simulink model "impmodel"  (R2023a)
settings: Solver=FixedStepDiscrete  StartTime=0.0  StopTime=8  RelTol=1e-3  EnableMultiTasking=on
values from neighbouring files (symbols this model uses):
  availableSpeedModes = 3    [params_f2838.mat]
  inverter_DRV8300 =     [params_f2838.mat]
  PI_params =     [params_f2838.mat]
  pmsm_ECI6360 =     [params_f2838.mat]
  PU_System =     [params_f2838.mat]
  target_f2838 =     [params_f2838.mat]
  Ts = 5e-05    [params_f2838.mat]
  Ts_motor = 2.5e-05    [params_f2838.mat]
  Ts_simulink = 2.5e-05    [params_f2838.mat]
  Ts_speed = 0.0005    [params_f2838.mat]
undefined symbols (not defined in the file or in its folder): Down, GPTRIP1SEL, TZ1, Up
libraries: simulink x35, c2802xlib x11, idelinklib_common x8, procinterlib x8, mcbcontrolslib x8, c280xlib x7, mcbpositiondecoderlib x7, slpidlib x5, svdschedulerlib x4, c2838xlib x2, autolibpmsminterior x1, mcbplantlib x1
(part 2 of 4)

== system impmodel/Input Controller/SpeedCommand_CodeGen ==
  note: This Subsystem is essential due to the fact that the voltage at the potentiometer will not reach 3.3 V.
      | At an ADC value bigger than 4000 the output will jump to 4095 (full speed)
  ADC1 : c2802xlib/ADC  blkParamProc=C2000_Type4  ADCModule=A  samplingMode=Single sample mode  ADCResolution=12-bit (Single-ended input)  useSOC1=SOC2  useSOC2=SOC0_SOC1  SOCAcquisitionWindow=7  SOCTriggerSource=Software  SOCInterruptTrigger=No ADCINT  Ts=0.01  dType=uint16  postInterrupt=off  interruptSel=ADCINT1  ADCINTContinuous=on  endma=off  chdma=1  conv1=ADCINA0  conv2=ADCINA0 and ADCINB0  conv1_Type4=ADCIN0  conv2_Type4=ADCIN0 and ADCIN1
      settings: LibrarySourceBlock=c2838xlib/ADC
  Check for SpeedRef : Subsystem
  normalizeADCValue : Gain  Gain=1/4095  OutDataTypeStr=fixdt(1,32,17)  RndMeth=Ceiling
  Speed_Ref : Outport
  wires:
  normalizeADCValue/1 -> Speed_Ref/1
  Check for SpeedRef/1(Out1) -> normalizeADCValue/1
  ADC1/1 -> Check for SpeedRef/1(In1)

== system impmodel/Input Controller/Subsystem ==
  ADC1 : c2802xlib/ADC  blkParamProc=C2000_Type4  ADCModule=C  samplingMode=Single sample mode  ADCResolution=12-bit (Single-ended input)  useSOC1=SOC5  useSOC2=SOC0_SOC1  SOCAcquisitionWindow=15  SOCTriggerSource=Software  SOCInterruptTrigger=No ADCINT  Ts=0.2  dType=uint16  postInterrupt=off  interruptSel=ADCINT1  ADCINTContinuous=on  endma=off  chdma=1  conv1=ADCINA0  conv2=ADCINA0 and ADCINB0  conv1_Type4=ADCIN2  conv2_Type4=ADCIN0 and ADCIN1
      settings: LibrarySourceBlock=c2838xlib/ADC
  Constant2 : Constant  Value=500e-3  OutDataTypeStr=fixdt(1,32,17)  SampleTime=-1
  Constant3 : Constant  Value=0.01  OutDataTypeStr=fixdt(1,32,17)  SampleTime=-1
  Divide : Product  Inputs=*/  OutDataTypeStr=fixdt(1,32,17)
  Gain : Gain  Gain=3.3/4095  OutDataTypeStr=fixdt(1,32,17)
  Subtract1 : Sum  Inputs=+-  OutDataTypeStr=fixdt(1,32,17)
  TCP_temp : Subsystem
  temperatureMOS : Outport
  wires:
  Constant3/1 -> Divide/2
  Gain/1 -> Subtract1/1
  Divide/1 -> TCP_temp/1(In1), temperatureMOS/1
  Constant2/1 -> Subtract1/2
  Subtract1/1 -> Divide/1
  ADC1/1 -> Gain/1

== system impmodel/Input Controller/speedMode_CodeGen ==
  Data Type Conversion : DataTypeConversion  OutDataTypeStr=fixdt(1,32,17)  SaturateOnIntegerOverflow=off  RndMeth=Floor
  Select first element : Selector  InputPortWidth=4  IndexOptions=Index vector (dialog)  Indices=[1]  OutputSizes=1
  Terminator : Terminator
  eCAN Receive1 : c280xlib/eCAN Receive  chipFamily=C280x  useModule=eCAN_A  mailboxNo=15  messageID=hex2dec('102')  messageType=Standard (11-bit identifier)  enableAcceptanceFiltering=off  messageIDMask=0  sampleTime=0.2  dataType=uint16  outputAction=Output last received values  initValue=0  outputMessageID=off  outputMessageLength=off  outputMessageTimeStamp=off  postInterrupt=off  interruptLine=0
      settings: LibrarySourceBlock=c28004xlib/eCAN Receive
  limit modes between 1 and 'availableSpeedModes' : Saturate  UpperLimit=availableSpeedModes  LowerLimit=1
  speedMode_CodeGen : Outport
  wires:
  eCAN Receive1/2 -> Select first element/1
  eCAN Receive1/1 -> Terminator/1
  Select first element/1 -> Data Type Conversion/1
  Data Type Conversion/1 -> limit modes between 1 and 'availableSpeedModes'/1
  limit modes between 1 and 'availableSpeedModes'/1 -> speedMode_CodeGen/1

== system impmodel/Inverter and Motor - Plant Model/Codegeneration ==
  Duty_Cycles : Inport
  Ground : Ground
  Ground1 : Ground
  Terminator : Terminator
  Iab_fb_Sim : Outport  VectorParamsAs1DForOutWhenUnconnected=off
  Pos_fb_Sim : Outport  Port=2  VectorParamsAs1DForOutWhenUnconnected=off
  wires:
  Duty_Cycles/1 -> Terminator/1
  Ground/1 -> Iab_fb_Sim/1
  Ground1/1 -> Pos_fb_Sim/1

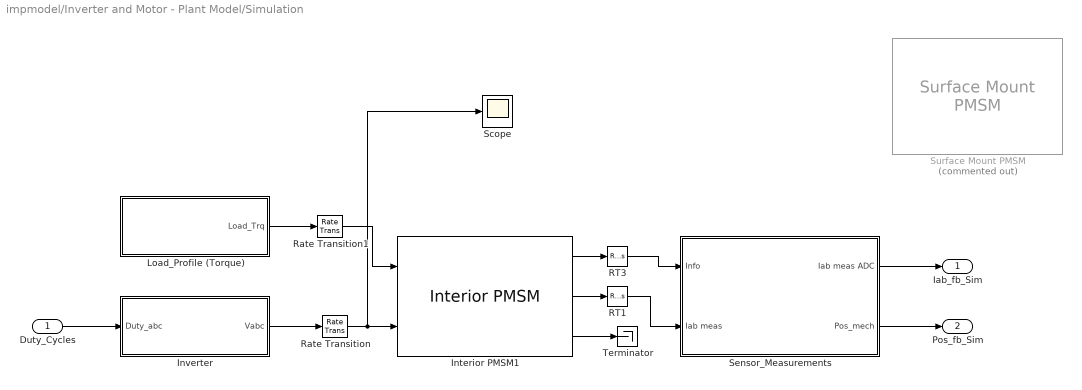
== system impmodel/Inverter and Motor - Plant Model/Simulation ==
  Duty_Cycles : Inport
  Interior PMSM1 : autolibpmsminterior/Interior PMSM  port_config=Torque  sim_type=Discrete  Ts=Ts_motor  P=pmsm_ECI6360.p  Rs=pmsm_ECI6360.Rs  Ldq=[pmsm_ECI6360.Ld, pmsm_ECI6360.Lq]  KConstText=Permanent flux linkage constant (lambda_pm):  lambda_pm=pmsm_ECI6360.FluxPM  Ke=pmsm_ECI6360.Ke  mechanical=[pmsm_ECI6360.J,0,0]  idq0=[0 0]  theta_init=0  omega_init=0  KConst=pmsm_ECI6360.FluxPM  lambda_pm_calc=pmsm_ECI6360.FluxPM  Kt=0.07  RefBlkName='autolibpmsminterior/Interior PMSM'  aMode=5
      settings: LibrarySourceBlock=mcblib/Electrical Systems/Motors/Interior PMSM
  Inverter : Subsystem
  Load_Profile (Torque) : Subsystem
  RT1 : RateTransition  Deterministic=off  OutPortSampleTime=Ts_simulink
  RT3 : RateTransition  Deterministic=off  OutPortSampleTime=Ts_simulink
  Rate Transition : RateTransition  Deterministic=off  OutPortSampleTime=Ts_motor
  Rate Transition1 : RateTransition  Deterministic=off  OutPortSampleTime=Ts_motor
  Scope : Scope
  Sensor_Measurements : Subsystem
  Surface Mount PMSM : autolibpmsmexterior/Surface Mount PMSM  Commented=on  port_config=Torque  sim_type=Discrete  Ts=Ts_motor  P=4  Rs=1  Ldq_=pmsm_ECI6360.Ld  KConstText=Permanent flux linkage constant (lambda_pm):  lambda_pm=0.039  Ke=pmsm_ECI6360.Ke  Kt=1.323  mechanical=[pmsm_ECI6360.J, pmsm_ECI6360.B, 0]  idq0=[0 0]  theta_init=0  omega_init=0  KConst=0.039  lambda_pm_calc=0.039  RefBlkName='autolibpmsmexterior/Surface Mount PMSM'  aMode=5  Ldq="[0.0002      0.0002]"
  Terminator : Terminator
  Iab_fb_Sim : Outport  VectorParamsAs1DForOutWhenUnconnected=off
  Pos_fb_Sim : Outport  Port=2  VectorParamsAs1DForOutWhenUnconnected=off
  wires:
  Sensor_Measurements/1(Iab meas ADC) -> Iab_fb_Sim/1
  Sensor_Measurements/2(Pos_mech) -> Pos_fb_Sim/1
  RT3/1 -> Sensor_Measurements/1(Info)
  Rate Transition1/1 -> Interior PMSM1/1
  RT1/1 -> Sensor_Measurements/2(Iab meas)
  Load_Profile (Torque)/1(Load_Trq) -> Rate Transition1/1
  Interior PMSM1/1 -> RT3/1
  Interior PMSM1/2 -> RT1/1
  Interior PMSM1/3 -> Terminator/1
  Rate Transition/1 -> Scope/1, Interior PMSM1/2
  Duty_Cycles/1 -> Inverter/1(Duty_abc)
  Inverter/1(Vabc) -> Rate Transition/1

== system impmodel/Speed Control/Digital_Freemode_Check ==
  Undervoltage_Sig : Inport
  Freemode : Inport  Port=2
  hot_temp : Inport  Port=3
  Check if Freemode is enabled : simulink/Logic and Bit Operations/Compare To Constant  relop===  const=1  OutDataTypeStr=boolean
  Check if MOSFETs are too hot : simulink/Logic and Bit Operations/Compare To Constant  relop===  const=1  OutDataTypeStr=boolean
  Check if Undervoltage is achieved : simulink/Logic and Bit Operations/Compare To Constant  relop===  const=1  OutDataTypeStr=boolean
  OR : Logic  Operator=OR  Inputs=3  AllPortsSameDT=off  OutDataTypeStr=boolean
  "Freemode_Sig  " : Outport
  wires:
  Freemode/1 -> Check if Freemode is enabled/1
  Undervoltage_Sig/1 -> Check if Undervoltage is achieved/1
  Check if Undervoltage is achieved/1 -> OR/1
  Check if Freemode is enabled/1 -> OR/2
  hot_temp/1 -> Check if MOSFETs are too hot/1
  Check if MOSFETs are too hot/1 -> OR/3
  OR/1 -> "Freemode_Sig  "/1

== system impmodel/Speed Control/Mechanical_Freemode_Check ==
  Freemode_Sig_Dig : Inport
  SafeState : Inport  Port=2
  If : If  IfExpression=u1 ~= 1
  If Action Subsystem : Subsystem  TreatAsAtomicUnit=on
  If Action Subsystem1 : Subsystem  TreatAsAtomicUnit=on
  Merge : Merge
  Freemode_Sig : Outport
  wires:
  SafeState/1 -> If/1
  Merge/1 -> Freemode_Sig/1
  Freemode_Sig_Dig/1 -> If Action Subsystem1/1(Freemode_Sig_Dig)
  If Action Subsystem/1(Out1) -> Merge/1
  If/1 -> If Action Subsystem/Action
  If Action Subsystem1/1(Out1) -> Merge/2
  If/2 -> If Action Subsystem1/Action

== system impmodel/Speed Control/PI_Controller_Speed ==
  N_ref : Inport
  N_fb : Inport  Port=2
  "  FreemodeEnabled?" : Inport  Port=3
  "Essential, so error of PI controller isn't rising" : Switch  Criteria=u2 > Threshold  OutDataTypeStr=fixdt(1,32,17)  SaturateOnIntegerOverflow=off  InputSameDT=off
  PID Controller : slpidlib/PID Controller  Controller=PI  Form=Parallel  TimeDomain=Discrete-time  UseExternalTs=off  SampleTime=-1  IntegratorMethod=Forward Euler  FilterMethod=Forward Euler  ControllerParametersSource=internal  P=PI_params.Kp_speed  I=PI_params.Ki_speed_texas*Ts_speed  UseKiTs=on  D=0  N=100  UseFilter=on  TunerSelectOption=Transfer Function Based (PID Tuner App)  InitialConditionSource=internal  InitialConditionForIntegrator=0  InitialConditionForFilter=0  DifferentiatorICPrevScaledInput=0  ExternalReset=none  TrackingMode=off  Kt=1  LimitOutput=on  SatLimitsSource=internal  UpperSaturationLimit=1  LowerSaturationLimit=-0.5  LinearizeAsGain=on  AntiWindupMode=clamping  Kb=1  LimitIntegrator=off  UpperIntegratorSaturationLimit=inf  LowerIntegratorSaturationLimit=-inf  RndMeth=Nearest  POutMin=[]  POutMax=[]  IOutMin=[]  IOutMax=[]  DOutMin=[]  DOutMax=[]  NOutMin=[]  NOutMax=[]  SumOutMin=[]  SumOutMax=[]  SaturationOutMin=[]  SaturationOutMax=[]  PParamMin=[]  PParamMax=[]  IParamMin=[]  IParamMax=[]  DParamMin=[]  DParamMax=[]  NParamMin=[]  NParamMax=[]  KbParamMin=[]  KbParamMax=[]  KtParamMin=[]  KtParamMax=[]  KbOutMin=[]  KbOutMax=[]  KtOutMin=[]  KtOutMax=[]  IntegratorOutMin=[]  IntegratorOutMax=[]  FilterOutMin=[]  FilterOutMax=[]  SumI1OutMin=[]  SumI1OutMax=[]  SumI2OutMin=[]  SumI2OutMax=[]  SumI3OutMin=[]  SumI3OutMax=[]  SumI4OutMin=[]  SumI4OutMax=[]  SumDOutMin=[]  SumDOutMax=[]  DifferentiatorOutMin=[]  DifferentiatorOutMax=[]  FilterDiffOutCoefMin=[]  FilterDiffOutCoefMax=[]  ReciprocalOutMin=[]  ReciprocalOutMax=[]  SumDenOutMin=[]  SumDenOutMax=[]  SumNumOutMin=[]  SumNumOutMax=[]  DivideOutMin=[]  DivideOutMax=[]  UdiffTsProdOutMin=[]  UdiffTsProdOutMax=[]  NTsProdOutMin=[]  NTsProdOutMax=[]  UintegralTsProdOutMin=[]  UintegralTsProdOutMax=[]  UngainTsProdOutMin=[]  UngainTsProdOutMax=[]  ClampingZeroOutDataTypeStr=Inherit: Inherit via back propagation  ClampingZeroOutMin=[]  ClampingZeroOutMax=[]  FilterDenConstantOutDataTypeStr=Inherit: Inherit via back propagation  FilterDenConstantOutMin=[]  FilterDenConstantOutMax=[]  PCopyOutDataTypeStr=Inherit: Inherit via back propagation  PCopyOutMin=[]  PCopyOutMax=[]  NCopyOutDataTypeStr=Inherit: Inherit via back propagation  NCopyOutMin=[]  NCopyOutMax=[]  IntegratorContinuousStateAttributes=''  IntegratorStateMustResolveToSignalObject=off  IntegratorRTWStateStorageClass=Auto  FilterContinuousStateAttributes=''  FilterStateMustResolveToSignalObject=off  FilterRTWStateStorageClass=Auto  ParallelPVariant=InternalParameters  IdealPVariant=Disabled  IVariant=InternalParameters  DVariant=Disabled  IntegratorVariant=Discrete  SatVariant=Enabled  AWVariant=DiscClampingParallel  PCopyVariant=Disabled  TRVariant=Disabled  FdbkBlocksVariant=Forward  IdealPFdbkVariant=Disabled  SatFdbkVariant=Disabled  DerivativeFilterVariant=Disabled  NVariant=Disabled  NCopyVariant=Disabled_SignalSpec  FilterICVariant=Disabled  IntegratorICVariant=InternalICs  ExternalResetVariant=Disabled  TRSumVariant=Passthrough  SumFdbkVariant=Disabled  SumVariant=Sum_PI  TsampFilterVariant=InternalTs  TsampNgainVariant=Passthrough  TsampIntegralVariant=Disabled_SignalSpec  ExternalSaturationOutDataTypeStr=Inherit: Same as second input
  Saturation : Saturate  UpperLimit=0  LowerLimit=0
  Sum : Sum  Inputs=|+-  RndMeth=Round
  Iq_ref : Outport  VectorParamsAs1DForOutWhenUnconnected=off
  wires:
  N_ref/1 -> Saturation/1, "Essential, so error of PI controller isn't rising"/3
  N_fb/1 -> Sum/2
  PID Controller/1 -> Iq_ref/1
  "  FreemodeEnabled?"/1 -> "Essential, so error of PI controller isn't rising"/2
  Saturation/1 -> "Essential, so error of PI controller isn't rising"/1
  Sum/1 -> PID Controller/1
  "Essential, so error of PI controller isn't rising"/1 -> Sum/1

== system impmodel/Speed Control/Speed calculator ==
  Speed_Ref_PU : Inport
  speedMode : Inport  Port=2
  Gain : Gain  Gain=floor(PU_System.N_base/availableSpeedModes)  OutDataTypeStr=fixdt(1,32,17)  RndMeth=Ceiling
  Product : Product  OutDataTypeStr=fixdt(1,32,17)
  Subsystem : Subsystem  Commented=through
  rpm2PU : Gain  Gain=1/PU_System.N_base  OutMax=1  OutDataTypeStr=fixdt(1,32,17)
  N_Ref : Outport
  wires:
  Speed_Ref_PU/1 -> Gain/1
  Gain/1 -> Product/2
  speedMode/1 -> Product/1
  Product/1 -> rpm2PU/1
  rpm2PU/1 -> Subsystem/1(In1)
  Subsystem/1(Out1) -> N_Ref/1

== system impmodel/Speed Control/TCP_SpeedRef ==
  In1 : Inport
  Data_Type_Fixed_Point : Subsystem  VariantControl=~isequal(dataType,'single')
  Interprocess Data Write : procinterlib/Interprocess Data Write  showPort=off  ChannelNum=6  NumBuff=1  IsIntEnabled=1  EnInterrupt=on  IPCBetween=1  CurrentPU=0  DataType=uint8  PartCores=CPU1<->CM  TargetType=0  ClientPU=TriCore1  ClientIntPrio=50
  wires:
  Data_Type_Fixed_Point/1(Data_Log) -> Interprocess Data Write/1
  In1/1 -> Data_Type_Fixed_Point/1(In1)

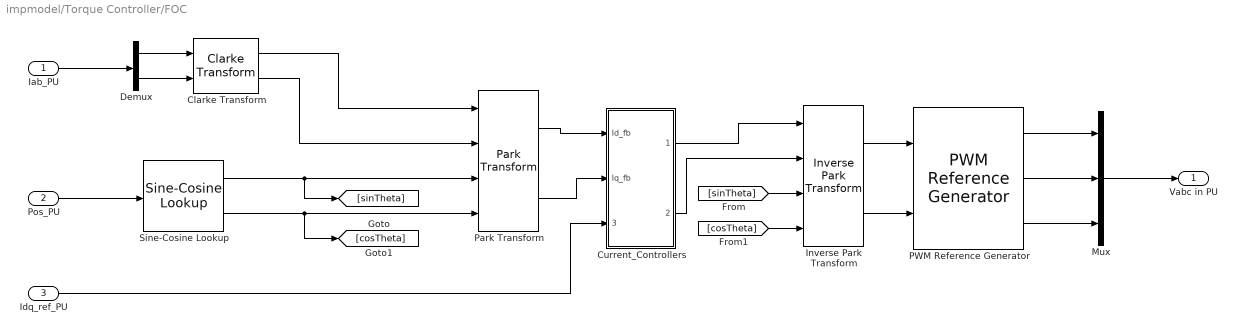
== system impmodel/Torque Controller/FOC ==
  Iab_PU : Inport
  Pos_PU : Inport  Port=2
  Idq_ref_PU : Inport  Port=3
  Clarke Transform : mcbcontrolslib/Clarke Transform  VariantControl=Variant2
      settings: LibrarySourceBlock=mcbhdllib/Controls/Math Transforms/Clarke Transform
  Current_Controllers : Subsystem
  Demux : Demux  Outputs=2
  Inverse Park Transform : mcbcontrolslib/Inverse Park Transform  AxisAlignment=D-axis
      settings: LibrarySourceBlock=mcbhdllib/Controls/Math Transforms/Inverse Park Transform
  Mux : Mux  Inputs=3
  PWM Reference Generator : mcbcontrolslib/PWM Reference Generator  inSignal=Valphabeta  modType=SVM: space vector modulation
      settings: LibrarySourceBlock=mcblib/Controls/Math Transforms/PWM Reference Generator
  Park Transform : mcbcontrolslib/Park Transform  AxisAlignment=D-axis
      settings: LibrarySourceBlock=mcbhdllib/Controls/Math Transforms/Park Transform
  Sine-Cosine Lookup : mcbcontrolslib/Sine-Cosine Lookup  AngleInput=Per-unit  N_points=1024
      settings: LibrarySourceBlock=mcblib/Controls/Math Transforms/Sine-Cosine Lookup
  Vabc in PU : Outport
  wires:
  Iab_PU/1 -> Demux/1
  Demux/1 -> Clarke Transform/1
  Demux/2 -> Clarke Transform/2
  Clarke Transform/1 -> Park Transform/1
  Clarke Transform/2 -> Park Transform/2
  Sine-Cosine Lookup/1 -> [sinTheta], Park Transform/3
  Sine-Cosine Lookup/2 -> [cosTheta], Park Transform/4
  Park Transform/1 -> Current_Controllers/1(Id_fb)
  Park Transform/2 -> Current_Controllers/2(Iq_fb)
  Idq_ref_PU/1 -> Current_Controllers/3(Idq_ref_PU)
  [sinTheta] -> Inverse Park Transform/3
  [cosTheta] -> Inverse Park Transform/4
  Inverse Park Transform/1 -> PWM Reference Generator/1
  Inverse Park Transform/2 -> PWM Reference Generator/2
  PWM Reference Generator/1 -> Mux/1
  PWM Reference Generator/2 -> Mux/2
  PWM Reference Generator/3 -> Mux/3
  Mux/1 -> Vabc in PU/1
  Pos_PU/1 -> Sine-Cosine Lookup/1
  Current_Controllers/1(Vd_ref) -> Inverse Park Transform/1
  Current_Controllers/2(Vq_ref) -> Inverse Park Transform/2

== system impmodel/Torque Controller/Iab_Meas_ADC ==
  ADC : c2802xlib/ADC  blkParamProc=C2000_Type4  ADCModule=B  samplingMode=Single sample mode  ADCResolution=12-bit (Single-ended input)  useSOC1=SOC0  useSOC2=SOC0_SOC1  SOCAcquisitionWindow=13  SOCTriggerSource=ePWM6_ADCSOCA  SOCInterruptTrigger=No ADCINT  Ts=-1  dType=uint16  postInterrupt=off  interruptSel=ADCINT1  ADCINTContinuous=on  endma=off  chdma=1  conv1=ADCINA0  conv2=ADCINA0 and ADCINB0  conv1_Type4=ADCIN0  conv2_Type4=ADCIN0 and ADCIN1
      settings: LibrarySourceBlock=c2838xlib/ADC
  ADC1 : c2802xlib/ADC  blkParamProc=C2000_Type4  ADCModule=B  samplingMode=Single sample mode  ADCResolution=12-bit (Single-ended input)  useSOC1=SOC1  useSOC2=SOC0_SOC1  SOCAcquisitionWindow=13  SOCTriggerSource=ePWM6_ADCSOCA  SOCInterruptTrigger=No ADCINT  Ts=-1  dType=uint16  postInterrupt=on  interruptSel=ADCINT1  ADCINTContinuous=on  endma=off  chdma=1  conv1=ADCINA0  conv2=ADCINA0 and ADCINB0  conv1_Type4=ADCIN2  conv2_Type4=ADCIN0 and ADCIN1
      settings: LibrarySourceBlock=c2838xlib/ADC
  Mux : Mux  Inputs=2
  Iab_ADC : Outport
  wires:
  Mux/1 -> Iab_ADC/1
  ADC/1 -> Mux/1
  ADC1/1 -> Mux/2

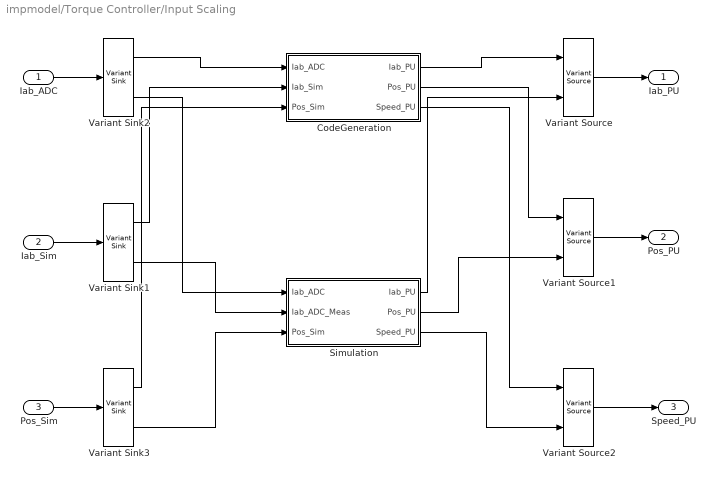
== system impmodel/Torque Controller/Input Scaling ==
  Iab_ADC : Inport
  Iab_Sim : Inport  Port=2
  Pos_Sim : Inport  Port=3
  CodeGeneration : Subsystem
  Simulation : Subsystem
  Variant Sink1 : VariantSink  VariantControlMode=sim codegen switching
  Variant Sink2 : VariantSink  VariantControlMode=sim codegen switching
  Variant Sink3 : VariantSink  VariantControlMode=sim codegen switching
  Variant Source : VariantSource  VariantControlMode=sim codegen switching
  Variant Source1 : VariantSource  VariantControlMode=sim codegen switching
  Variant Source2 : VariantSource  VariantControlMode=sim codegen switching
  Iab_PU : Outport
  Pos_PU : Outport  Port=2
  Speed_PU : Outport  Port=3
  wires:
  Pos_Sim/1 -> Variant Sink3/1
  Iab_Sim/1 -> Variant Sink1/1
  Iab_ADC/1 -> Variant Sink2/1
  Variant Sink2/1 -> CodeGeneration/1(Iab_ADC)
  Variant Sink1/1 -> CodeGeneration/2(Iab_Sim)
  Variant Sink3/1 -> CodeGeneration/3(Pos_Sim)
  Variant Sink2/2 -> Simulation/1(Iab_ADC)
  Variant Sink1/2 -> Simulation/2(Iab_ADC_Meas)
  Variant Sink3/2 -> Simulation/3(Pos_Sim)
  CodeGeneration/1(Iab_PU) -> Variant Source/1
  Simulation/1(Iab_PU) -> Variant Source/2
  CodeGeneration/2(Pos_PU) -> Variant Source1/1
  Simulation/2(Pos_PU) -> Variant Source1/2
  Simulation/3(Speed_PU) -> Variant Source2/2
  CodeGeneration/3(Speed_PU) -> Variant Source2/1
  Variant Source/1 -> Iab_PU/1
  Variant Source1/1 -> Pos_PU/1
  Variant Source2/1 -> Speed_PU/1

== system impmodel/Torque Controller/Output ==
  Scaled_DC : Inport
  CodeGeneration : Subsystem
  Scope : Scope
  Simulation : Subsystem
  Variant Sink : VariantSink  VariantControlMode=sim codegen switching
  Duty Cycle : Outport
  wires:
  Scaled_DC/1 -> Variant Sink/1
  Simulation/1(Output) -> Scope/1, Duty Cycle/1
  Variant Sink/1 -> CodeGeneration/1(In1)
  Variant Sink/2 -> Simulation/1(Input)

== system impmodel/Torque Controller/PWM1 ==
  Scaled_DC_PWM1 : Inport
  Freemode_Sig : Inport  Port=2
  Constant : Constant  Value=0  OutDataTypeStr=fixdt(1,32,17)  SampleTime=-1
  Constant1 : Constant  OutDataTypeStr=fixdt(1,32,17)  SampleTime=-1
  Switch : Switch  Criteria=u2 > Threshold  SaturateOnIntegerOverflow=off  InputSameDT=off  OutDataTypeStr=Inherit: Same as first input
  Switch1 : Switch  Criteria=u2 > Threshold  SaturateOnIntegerOverflow=off  InputSameDT=off  OutDataTypeStr=Inherit: Same as first input
  WA : Outport
  WB : Outport  Port=2
  wires:
  Freemode_Sig/1 -> Switch1/2, Switch/2
  Switch/1 -> WA/1
  Switch1/1 -> WB/1
  Scaled_DC_PWM1/1 -> Switch/3, Switch1/3
  Constant/1 -> Switch/1
  Constant1/1 -> Switch1/1

== system impmodel/Torque Controller/PWM2 ==
  Scaled_DC_PWM2 : Inport
  Freemode_Sig : Inport  Port=2
  Constant : Constant  Value=0  OutDataTypeStr=fixdt(1,32,17)  SampleTime=-1
  Constant1 : Constant  OutDataTypeStr=fixdt(1,32,17)  SampleTime=-1
  Switch : Switch  Criteria=u2 > Threshold  SaturateOnIntegerOverflow=off  InputSameDT=off  OutDataTypeStr=Inherit: Same as first input
  Switch1 : Switch  Criteria=u2 > Threshold  SaturateOnIntegerOverflow=off  InputSameDT=off  OutDataTypeStr=Inherit: Same as first input
  WA : Outport
  WB : Outport  Port=2
  wires:
  Switch/1 -> WA/1
  Switch1/1 -> WB/1
  Constant/1 -> Switch/1
  Freemode_Sig/1 -> Switch/2, Switch1/2
  Constant1/1 -> Switch1/1
  Scaled_DC_PWM2/1 -> Switch1/3, Switch/3

== system impmodel/Torque Controller/PWM3 ==
  Scaled_DC_PWM3 : Inport
  Freemode_Sig : Inport  Port=2
  Constant : Constant  Value=0  OutDataTypeStr=fixdt(1,32,17)  SampleTime=-1
  Constant1 : Constant  OutDataTypeStr=fixdt(1,32,17)  SampleTime=-1
  Switch : Switch  Criteria=u2 > Threshold  SaturateOnIntegerOverflow=off  InputSameDT=off  OutDataTypeStr=Inherit: Same as first input
  Switch1 : Switch  Criteria=u2 > Threshold  SaturateOnIntegerOverflow=off  InputSameDT=off  OutDataTypeStr=Inherit: Same as first input
  WA : Outport
  WB : Outport  Port=2
  wires:
  Switch/1 -> WA/1
  Switch1/1 -> WB/1
  Constant/1 -> Switch/1
  Freemode_Sig/1 -> Switch1/2, Switch/2
  Constant1/1 -> Switch1/1
  Scaled_DC_PWM3/1 -> Switch1/3, Switch/3

== system impmodel/Torque Controller/Scaling DutyCycles ==
  Unscaled_DC : Inport
  CodeGen : Subsystem
  Demux : Demux  Outputs=3
  Sim : Subsystem
  Variant Sink : VariantSink  VariantControlMode=sim codegen switching
  Variant Source : VariantSource  VariantControlMode=sim codegen switching
  Scaled_DC_PWM1 : Outport
  Scaled_DC_PWM2 : Outport  Port=2
  Scaled_DC_PWM3 : Outport  Port=3
  wires:
  Demux/1 -> Scaled_DC_PWM1/1
  Demux/2 -> Scaled_DC_PWM2/1
  Demux/3 -> Scaled_DC_PWM3/1
  Variant Source/1 -> Demux/1
  Unscaled_DC/1 -> Variant Sink/1
  Sim/1(Out1) -> Variant Source/2
  Variant Sink/2 -> Sim/1(In1)
  Variant Sink/1 -> CodeGen/1(In1)
  CodeGen/1(Out1) -> Variant Source/1

== system impmodel/Torque Controller/TCP_Position ==
  In1 : Inport
  Data_Type_Fixed_Point : Subsystem  VariantControl=~isequal(dataType,'single')
  Interprocess Data Write : procinterlib/Interprocess Data Write  showPort=off  ChannelNum=0  NumBuff=1  IsIntEnabled=1  EnInterrupt=on  IPCBetween=1  CurrentPU=0  DataType=uint8  PartCores=CPU1<->CM  TargetType=0  ClientPU=TriCore1  ClientIntPrio=50
  wires:
  Data_Type_Fixed_Point/1(Data_Log) -> Interprocess Data Write/1
  In1/1 -> Data_Type_Fixed_Point/1(In1)

== system impmodel/Torque Controller/TCP_Speed ==
  " " : Inport
  Data_Type_Fixed_Point : Subsystem  VariantControl=~isequal(dataType,'single')
  Interprocess Data Write : procinterlib/Interprocess Data Write  showPort=off  ChannelNum=1  NumBuff=1  IsIntEnabled=1  EnInterrupt=on  IPCBetween=1  CurrentPU=0  DataType=uint8  PartCores=CPU1<->CM  TargetType=0  ClientPU=TriCore1  ClientIntPrio=50
  wires:
  Data_Type_Fixed_Point/1(Data_Log) -> Interprocess Data Write/1
  " "/1 -> Data_Type_Fixed_Point/1(In1)

== system impmodel/ADC Offset Function/Calculate ADC Offset /For Iterator Subsystem ==
  ADC_B_IN0 : c2802xlib/ADC  Priority=20  blkParamProc=C2000_Type4  ADCModule=B  samplingMode=Single sample mode  ADCResolution=12-bit (Single-ended input)  useSOC1=SOC2  useSOC2=SOC0_SOC1  SOCAcquisitionWindow=15  SOCTriggerSource=Software  SOCInterruptTrigger=No ADCINT  Ts=-1  dType=uint16  postInterrupt=off  interruptSel=ADCINT1  ADCINTContinuous=on  endma=off  chdma=1  conv1=ADCINA0  conv2=ADCINA0 and ADCINB0  conv1_Type4=ADCIN0  conv2_Type4=ADCIN0 and ADCIN1
  ADC_B_IN2 : c2802xlib/ADC  Priority=20  blkParamProc=C2000_Type4  ADCModule=B  samplingMode=Single sample mode  ADCResolution=12-bit (Single-ended input)  useSOC1=SOC3  useSOC2=SOC0_SOC1  SOCAcquisitionWindow=15  SOCTriggerSource=Software  SOCInterruptTrigger=No ADCINT  Ts=-1  dType=uint16  postInterrupt=off  interruptSel=ADCINT1  ADCINTContinuous=on  endma=off  chdma=1  conv1=ADCINA0  conv2=ADCINA0 and ADCINB0  conv1_Type4=ADCIN2  conv2_Type4=ADCIN0 and ADCIN1
  For Iterator : ForIterator  IterationLimit=16  IterationVariableDataType=uint16
  If : If  IfExpression=u1 > 8  ShowElse=off
  If Action Subsystem : Subsystem  TreatAsAtomicUnit=on
  Out1 : Outport
  Out2 : Outport  Port=2
  wires:
  For Iterator/1 -> If/1
  ADC_B_IN0/1 -> If Action Subsystem/1(In1)
  ADC_B_IN2/1 -> If Action Subsystem/2(In2)
  If Action Subsystem/1(Out1) -> Out1/1
  If Action Subsystem/2(Out2) -> Out2/1
  If/1 -> If Action Subsystem/Action

== system impmodel/ADC Offset Function/Calculate ADC Offset /If Action Subsystem ==
  In1 : Inport
  Action Port : ActionPort  ActionPortLabel=if(u1 > u3 & u1 < u2)
  Data Store Write1 : DataStoreWrite  DataStoreName=IaOffset  IndexOptions=Index vector (dialog)  Indices=1  OutputSizes=1
  wires:
  In1/1 -> Data Store Write1/1

== system impmodel/ADC Offset Function/Calculate ADC Offset /If Action Subsystem1 ==
  Action Port : ActionPort  ActionPortLabel=else
  Constant : Constant  Value=inverter_DRV8300.CtSensAOffset  OutDataTypeStr=Inherit: Inherit via back propagation
  Data Store Write1 : DataStoreWrite  DataStoreName=IaOffset  IndexOptions=Index vector (dialog)  Indices=1  OutputSizes=1
  wires:
  Constant/1 -> Data Store Write1/1

== system impmodel/ADC Offset Function/Calculate ADC Offset /If Action Subsystem2 ==
  In1 : Inport
  Action Port : ActionPort  ActionPortLabel=if(u1 > u3 & u1 < u2)
  Data Store Write2 : DataStoreWrite  DataStoreName=IbOffset  IndexOptions=Index vector (dialog)  Indices=1  OutputSizes=1
  wires:
  In1/1 -> Data Store Write2/1

== system impmodel/ADC Offset Function/Calculate ADC Offset /If Action Subsystem3 ==
  Action Port : ActionPort  ActionPortLabel=else
  Constant1 : Constant  Value=inverter_DRV8300.CtSensBOffset  OutDataTypeStr=Inherit: Inherit via back propagation
  Data Store Write2 : DataStoreWrite  DataStoreName=IbOffset  IndexOptions=Index vector (dialog)  Indices=1  OutputSizes=1
  wires:
  Constant1/1 -> Data Store Write2/1

== system impmodel/Hall Sensor A/Capture Event Selection/Output 0 ==
  Action Port : ActionPort  ActionPortLabel=else
  Constant : Constant  Value=0  OutDataTypeStr=boolean  SampleTime=-1
  Out1 : Outport
  wires:
  Constant/1 -> Out1/1

== system impmodel/Hall Sensor A/Capture Event Selection/Output 1 ==
  Action Port : ActionPort  ActionPortLabel=if((u1 == 5 | u1 == 3))
  Constant : Constant  OutDataTypeStr=boolean  SampleTime=-1
  Out1 : Outport
  wires:
  Constant/1 -> Out1/1

== system impmodel/Hall Sensor B/Capture Event Selection/Output 0 ==
  Action Port : ActionPort  ActionPortLabel=else
  Constant : Constant  Value=0  OutDataTypeStr=boolean  SampleTime=-1
  Out1 : Outport
  wires:
  Constant/1 -> Out1/1

== system impmodel/Hall Sensor B/Capture Event Selection/Output 1 ==
  Action Port : ActionPort  ActionPortLabel=if((u1 == 3 | u1 == 6))
  Constant : Constant  OutDataTypeStr=boolean  SampleTime=-1
  Out1 : Outport
  wires:
  Constant/1 -> Out1/1

== system impmodel/Hall Sensor C/Capture Event Selection/Output 0 ==
  Action Port : ActionPort  ActionPortLabel=else
  Constant : Constant  Value=0  OutDataTypeStr=boolean  SampleTime=-1
  Out1 : Outport
  wires:
  Constant/1 -> Out1/1

== system impmodel/Hall Sensor C/Capture Event Selection/Output 1 ==
  Action Port : ActionPort  ActionPortLabel=if((u1 == 5 | u1 == 6))
  Constant : Constant  OutDataTypeStr=boolean  SampleTime=-1
  Out1 : Outport
  wires:
  Constant/1 -> Out1/1

== system impmodel/IPC Write for eCAP INTs/TCP_HallA/Data_Type_Fixed_Point ==
  In1 : Inport
  Data Type Conversion3 : DataTypeConversion  OutDataTypeStr=uint32  ConvertRealWorld=Stored Integer (SI)  RndMeth=Simplest  SaturateOnIntegerOverflow=off
  Data_Log : Outport
  wires:
  Data Type Conversion3/1 -> Data_Log/1
  In1/1 -> Data Type Conversion3/1

== system impmodel/IPC Write for eCAP INTs/TCP_HallB/Data_Type_Fixed_Point ==
  In1 : Inport
  Data Type Conversion3 : DataTypeConversion  OutDataTypeStr=uint32  ConvertRealWorld=Stored Integer (SI)  RndMeth=Simplest  SaturateOnIntegerOverflow=off
  Data_Log : Outport
  wires:
  In1/1 -> Data Type Conversion3/1
  Data Type Conversion3/1 -> Data_Log/1

== system impmodel/IPC Write for eCAP INTs/TCP_HallC/Data_Type_Fixed_Point ==
  In1 : Inport
  Data Type Conversion3 : DataTypeConversion  OutDataTypeStr=uint32  ConvertRealWorld=Stored Integer (SI)  RndMeth=Simplest  SaturateOnIntegerOverflow=off
  Data_Log : Outport
  wires:
  Data Type Conversion3/1 -> Data_Log/1
  In1/1 -> Data Type Conversion3/1

== system impmodel/IPC Write for eCAP INTs/TCP_HallState/Data_Type_Fixed_Point ==
  In1 : Inport
  Data Type Conversion3 : DataTypeConversion  OutDataTypeStr=uint32  ConvertRealWorld=Stored Integer (SI)  RndMeth=Simplest  SaturateOnIntegerOverflow=off
  Data_Log : Outport
  wires:
  In1/1 -> Data Type Conversion3/1
  Data Type Conversion3/1 -> Data_Log/1

== system impmodel/Input Controller/SpeedCommand_CodeGen/Check for SpeedRef ==
  In1 : Inport
  If : If  IfExpression=u1 > 4000
  If Action Subsystem : Subsystem  TreatAsAtomicUnit=on
  If Action Subsystem1 : Subsystem  TreatAsAtomicUnit=on
  Merge : Merge
  Out1 : Outport
  wires:
  In1/1 -> If Action Subsystem1/1(In1), If/1
  Merge/1 -> Out1/1
  If/1 -> If Action Subsystem/Action
  If/2 -> If Action Subsystem1/Action
  If Action Subsystem/1(Out1) -> Merge/1
  If Action Subsystem1/1(Out1) -> Merge/2

== system impmodel/Input Controller/Subsystem/TCP_temp ==
  In1 : Inport
  Data_Type_Fixed_Point : Subsystem  VariantControl=~isequal(dataType,'single')
  Interprocess Data Write : procinterlib/Interprocess Data Write  showPort=off  ChannelNum=7  NumBuff=1  IsIntEnabled=1  EnInterrupt=on  IPCBetween=1  CurrentPU=0  DataType=uint8  PartCores=CPU1<->CM  TargetType=0  ClientPU=TriCore1  ClientIntPrio=50
  wires:
  Data_Type_Fixed_Point/1(Data_Log) -> Interprocess Data Write/1
  In1/1 -> Data_Type_Fixed_Point/1(In1)

== system impmodel/Inverter and Motor - Plant Model/Simulation/Inverter ==
  Duty_abc : Inport
  Average-Value Inverter : mcbplantlib/Average-Value Inverter
  Constant2 : Constant  Value=inverter_DRV8300.V_dc  OutDataTypeStr=single  SampleTime=-1
  Data Type Conversion1 : DataTypeConversion  OutDataTypeStr=single  RndMeth=Simplest  SaturateOnIntegerOverflow=off
  Rate Transition3 : RateTransition  Integrity=off  OutPortSampleTime=Ts_inverter
  Vabc : Outport  VectorParamsAs1DForOutWhenUnconnected=off
  wires:
  Duty_abc/1 -> Data Type Conversion1/1
  Data Type Conversion1/1 -> Rate Transition3/1
  Rate Transition3/1 -> Average-Value Inverter/1
  Constant2/1 -> Average-Value Inverter/2
  Average-Value Inverter/1 -> Vabc/1

== system impmodel/Inverter and Motor - Plant Model/Simulation/Load_Profile (Torque) ==
  Data Type Conversion : DataTypeConversion  OutDataTypeStr=single  SaturateOnIntegerOverflow=off  RndMeth=Floor
  IIR Filter : mcbcontrolslib/IIR Filter  VariantControl=Low Pass Filter  VariantSelect=Low-pass  Filter_constant=0.01  advancedSettings=off  Ts=50e-6  cutOff_freq=32.1525
  T_load : Step  Time=5  Before=0.1*pmsm_ECI6360.T_rated  After=0.1*pmsm_ECI6360.T_rated  SampleTime=Ts_simulink
  Load_Trq : Outport  VectorParamsAs1DForOutWhenUnconnected=off
  wires:
  T_load/1 -> Data Type Conversion/1
  Data Type Conversion/1 -> IIR Filter/1
  IIR Filter/1 -> Load_Trq/1

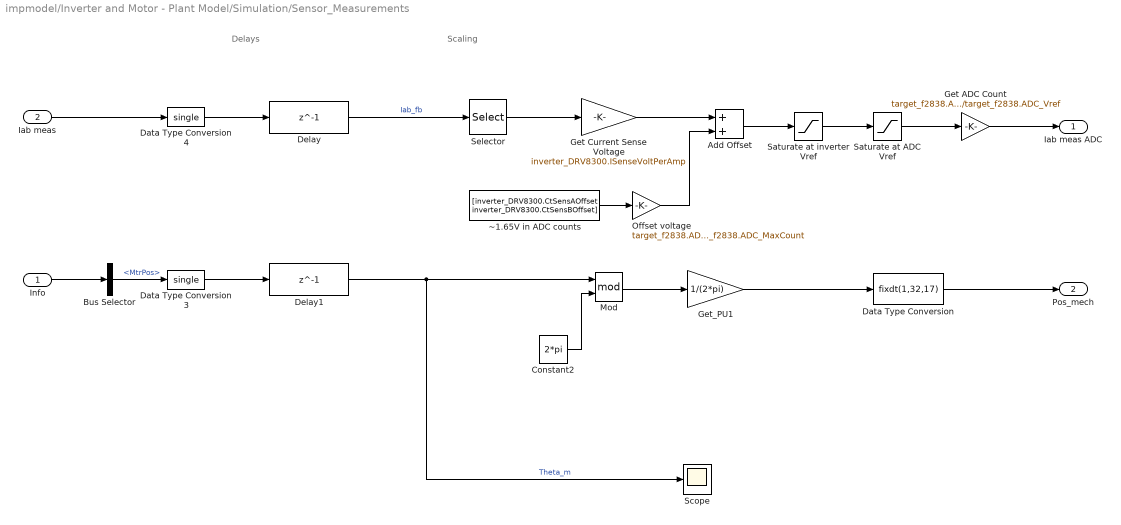
== system impmodel/Inverter and Motor - Plant Model/Simulation/Sensor_Measurements ==
  note: Scaling
  note: Delays
  Info : Inport
  Iab meas : Inport  Port=2
  Add Offset : Sum  RndMeth=Simplest
  Bus Selector : BusSelector  OutputSignals=MtrPos
  Constant2 : Constant  Value=2*pi  OutDataTypeStr=single  SampleTime=-1
  Data Type Conversion : DataTypeConversion  OutDataTypeStr=fixdt(1,32,17)  SaturateOnIntegerOverflow=off  RndMeth=Floor
  Data Type Conversion3 : DataTypeConversion  OutDataTypeStr=single  RndMeth=Simplest  SaturateOnIntegerOverflow=off
  Data Type Conversion4 : DataTypeConversion  OutDataTypeStr=single  RndMeth=Simplest  SaturateOnIntegerOverflow=off
  Delay : Delay  DelayLength=1
  Delay1 : Delay  DelayLength=1
  Get ADC Count : Gain  Gain=target_f2838.ADC_MaxCount/target_f2838.ADC_Vref  OutMin=0  OutMax=target_f2838.ADC_MaxCount  OutDataTypeStr=uint16  RndMeth=Simplest
  Get Current Sense Voltage : Gain  Gain=inverter_DRV8300.ISenseVoltPerAmp  RndMeth=Simplest  OutDataTypeStr=Inherit: Same as input
  Get_PU1 : Gain  Gain=1/(2*pi)  RndMeth=Simplest  OutDataTypeStr=Inherit: Same as input
  Mod : Math  Operator=mod
  Offset voltage : Gain  Gain=target_f2838.ADC_Vref / target_f2838.ADC_MaxCount  RndMeth=Simplest
  Saturate at ADC Vref : Saturate  UpperLimit=target_f2838.ADC_Vref  LowerLimit=0
  Saturate at inverter Vref : Saturate  UpperLimit=inverter_DRV8300.ISenseVref  LowerLimit=0
  Scope : Scope
  Selector : Selector  InputPortWidth=3  IndexOptions=Index vector (dialog)  Indices=[1 2]  OutputSizes=1
  ~1.65V in ADC counts : Constant  Value=[inverter_DRV8300.CtSensAOffset inverter_DRV8300.CtSensBOffset]  OutDataTypeStr=uint16  SampleTime=-1
  Iab meas ADC : Outport  VectorParamsAs1DForOutWhenUnconnected=off
  Pos_mech : Outport  Port=2
  wires:
  Delay/1 -> Selector/1  "Iab_fb"
  Data Type Conversion4/1 -> Delay/1
  Iab meas/1 -> Data Type Conversion4/1
  Info/1 -> Bus Selector/1
  Data Type Conversion3/1 -> Delay1/1
  Get_PU1/1 -> Data Type Conversion/1
  Bus Selector/1 -> Data Type Conversion3/1  "<MtrPos>"
  Constant2/1 -> Mod/2
  Mod/1 -> Get_PU1/1
  Delay1/1 -> Scope/1, Mod/1  "Theta_m"
  Selector/1 -> Get Current Sense Voltage/1
  Saturate at inverter Vref/1 -> Saturate at ADC Vref/1
  Add Offset/1 -> Saturate at inverter Vref/1
  Get ADC Count/1 -> Iab meas ADC/1
  Offset voltage/1 -> Add Offset/2
  Saturate at ADC Vref/1 -> Get ADC Count/1
  ~1.65V in ADC counts/1 -> Offset voltage/1
  Get Current Sense Voltage/1 -> Add Offset/1
  Data Type Conversion/1 -> Pos_mech/1

== system impmodel/Speed Control/Mechanical_Freemode_Check/If Action Subsystem ==
  Action Port : ActionPort  ActionPortLabel=if(u1 ~= 1)
  Constant : Constant  OutDataTypeStr=boolean  SampleTime=-1
  Out1 : Outport
  wires:
  Constant/1 -> Out1/1

== system impmodel/Speed Control/Mechanical_Freemode_Check/If Action Subsystem1 ==
  Freemode_Sig_Dig : Inport
  Action Port : ActionPort  ActionPortLabel=else
  Out1 : Outport
  wires:
  Freemode_Sig_Dig/1 -> Out1/1

== system impmodel/Speed Control/Speed calculator/Subsystem ==
  In1 : Inport
  Data Type Conversion : DataTypeConversion  OutDataTypeStr=single  SaturateOnIntegerOverflow=off  RndMeth=Floor
  If : If  IfExpression=u1 > 0.94
  If Action Subsystem : Subsystem  TreatAsAtomicUnit=on
  If Action Subsystem1 : Subsystem  TreatAsAtomicUnit=on
  Merge : Merge
  Out1 : Outport
  wires:
  In1/1 -> Data Type Conversion/1
  If/1 -> If Action Subsystem/Action
  If/2 -> If Action Subsystem1/Action
  Merge/1 -> Out1/1
  If Action Subsystem/1(Out1) -> Merge/1
  If Action Subsystem1/1(Out1) -> Merge/2
  Data Type Conversion/1 -> If Action Subsystem1/1(In1), If/1

== system impmodel/Speed Control/TCP_SpeedRef/Data_Type_Fixed_Point ==
  In1 : Inport
  Data Type Conversion : DataTypeConversion  OutDataTypeStr=fixdt(1,32,17)  RndMeth=Simplest  SaturateOnIntegerOverflow=off
  Data Type Conversion3 : DataTypeConversion  OutDataTypeStr=uint32  ConvertRealWorld=Stored Integer (SI)  RndMeth=Simplest  SaturateOnIntegerOverflow=off
  Data_Log : Outport
  wires:
  In1/1 -> Data Type Conversion/1
  Data Type Conversion3/1 -> Data_Log/1
  Data Type Conversion/1 -> Data Type Conversion3/1

== system impmodel/Torque Controller/FOC/Current_Controllers ==
  Id_fb : Inport
  Iq_fb : Inport  Port=2
  Idq_ref_PU : Inport  Port=3
  DQ Limiter : mcbcontrolslib/DQ Limiter  satMethodInputType=Specify via dialog  satMethodSelected=D-Q equivalence  satLimitInputType=Specify via dialog  Vmax=0.95
  Demux : Demux  Outputs=2
  PI_Controller_Id : Subsystem
  PI_Controller_Iq : Subsystem
  Sum : Sum  Inputs=|+-
  Sum1 : Sum  Inputs=|+-
  Terminator : Terminator
  Vd_ref : Outport  VectorParamsAs1DForOutWhenUnconnected=off
  Vq_ref : Outport  Port=2  VectorParamsAs1DForOutWhenUnconnected=off
  wires:
  Iq_fb/1 -> Sum1/2
  Idq_ref_PU/1 -> Demux/1
  Demux/1 -> Sum/1  "Id_Ref"
  Demux/2 -> Sum1/1  "Iq_Ref"
  DQ Limiter/1 -> Vd_ref/1
  DQ Limiter/2 -> Vq_ref/1
  DQ Limiter/3 -> Terminator/1
  Sum/1 -> PI_Controller_Id/1(Id_in)
  Id_fb/1 -> Sum/2
  Sum1/1 -> PI_Controller_Iq/1(Iq_in)
  PI_Controller_Id/1(V_ref) -> DQ Limiter/1
  PI_Controller_Iq/1(V_ref) -> DQ Limiter/2

== system impmodel/Torque Controller/Input Scaling/CodeGeneration ==
  Iab_ADC : Inport
  Iab_Sim : Inport  Port=2
  Pos_Sim : Inport  Port=3
  Calculate Position from Hall : Subsystem  TreatAsAtomicUnit=on
  Convert ADC value to PU : Subsystem
  Terminator : Terminator
  Terminator1 : Terminator
  Iab_PU : Outport
  Pos_PU : Outport  Port=2
  Speed_PU : Outport  Port=3
  wires:
  Convert ADC value to PU/1(Iab_PU) -> Iab_PU/1
  Iab_ADC/1 -> Convert ADC value to PU/1(Iab_ADC)
  Calculate Position from Hall/1(Pos_PU) -> Pos_PU/1
  Iab_Sim/1 -> Terminator/1
  Pos_Sim/1 -> Terminator1/1
  Calculate Position from Hall/2(Speed_PU) -> Speed_PU/1

== system impmodel/Torque Controller/Input Scaling/Simulation ==
  Iab_ADC : Inport
  Iab_ADC_Meas : Inport  Port=2
  Pos_Sim : Inport  Port=3
  Convert Iab to PU : Subsystem
  Convert Pos to PU : Subsystem
  Terminator : Terminator
  Iab_PU : Outport
  Pos_PU : Outport  Port=2
  Speed_PU : Outport  Port=3
  wires:
  Iab_ADC/1 -> Terminator/1
  Convert Pos to PU/1(Theta) -> Pos_PU/1
  Convert Pos to PU/2(Speed_PU) -> Speed_PU/1
  Pos_Sim/1 -> Convert Pos to PU/1(Pos_Sim)
  Convert Iab to PU/1(Iab_PU) -> Iab_PU/1
  Iab_ADC_Meas/1 -> Convert Iab to PU/1(Iab_ADC_Sim)
